simulink model "KinarmStroopTask_260119"  (R2019b)
settings: Solver=ode4  StartTime=0.0  StopTime=inf  FixedStep=BKIN_STEP_TIME  RelTol=1e-3  EnableMultiTasking=on
StartFcn:
  |  warndlg('Dexterit-E models cannot run under simulation. Please compile your model and run it from within Dexterit-E.');set_param(bdroot,'SimulationCommand','stop')
model workspace (MAT data in the model file):
  BKIN_KINEMATIC_FRAME_SIZE = 400
  BKIN_STEP_TIME = 0.00025
  COLOUR_1 = 6
  COLOUR_2 = 7
  COLOUR_3 = 8
  COLOUR_4 = 9
  COLOUR_5 = 10
  E_CONG = 16
  E_CORRECT = 22
  E_FALSE_START = 28
  E_FIX_OFF = 33
  E_FIX_ON = 32
  E_INCONG = 17
  E_INCORRECT = 24
  E_NO_EVENT = 0
  E_REACHED_BLUE = 25
  E_REACHED_GREEN = 26
  E_REACHED_RED = 23
  E_REACHED_T1 = 18
  E_REACHED_T2 = 19
  E_REACHED_T3 = 20
  E_REACHED_T4 = 21
  E_REACHED_YELLOW = 27
  E_SCOL_BLUE = 13
  E_SCOL_GREEN = 14
  E_SCOL_RED = 12
  E_SCOL_YELLOW = 15
  E_STEXT_BLUE = 9
  E_STEXT_GREEN = 10
  E_STEXT_RED = 8
  E_STEXT_YELLOW = 11
  E_STROOP_OFF = 31
  E_T1_ON = 4
  E_T2_ON = 5
  E_T3_ON = 6
  E_T4_ON = 7
  E_TIMED_OUT = 29
  E_TRIAL_END = 30
  E_TRIAL_START = 3
  FIX_DELAY = 12
  FIX_ON_TIME = 11
  FIX_RAND = 13
  FIX_TARG_COL = 4
  FLICKER_ON = 9
  FLICKER_TIME = 10
  LENGTH = 3
  LOAD_X = 1
  LOAD_Y = 2
  PERTURB_SET = 9
  POSTRESP_DELAY = 3
  RADIUS_VIS = 3
  RAMP_DURATION = 4
  RAND_TEXTLOC = 8
  REACH_DELAY = 1
  REACH_RAND = 6
  REACH_TO = 7
  RESULT_TARG_COL = 3
  START_TARG_COL = 2
  STROKE_WIDTH = 13
  STROOP_TARG_COL = 1
  STROOP_USE = 5
  TARG_LENGTH = 3
  TARG_WIDTH = 4
  TEXT = 11
  TEXT1_TARG_COL = 5
  TEXT2_TARG_COL = 6
  TEXT3_TARG_COL = 7
  TEXT4_TARG_COL = 8
  TEXTCIRCLE_MOVE = 14
  TEXTSHOW_DELAY = 2
  TEXT_SIZE = 12
  WIDTH = 4
  Width = 4
  X_LENGTH = 4
  Y_LENGTH = 5
  col_x = 1
  col_y = 2
undefined symbols (not defined in the file or in its folder): slselsubs
libraries: Video x9, General x3, KINARM_general x2, KINARM_EP_loads x2
settings Model: ModifiedComment=chris -- Wed Feb 16 09:18:30 2005 -- Version 1.1384  ModifiedHistory=Feb 16/05 - Add error repeat, add offset ramp  ExtModeArmWhenConnect=off  ExtModeLogAll=off  OrderedModelArguments=off  Creator=Chris Grebeldinger  LastModifiedBy=apark2
settings SolverCC: AutoInsertRateTranBlk=on
settings DataIOCC: SaveFormat=Array  SignalLoggingSaveFormat=ModelDataLogs  SaveOutput=off  SaveTime=off  ReturnWorkspaceOutputs=off  SignalLoggingName=sigsOut
settings OptimizationCC: BlockReduction=off  BooleanDataType=off  OptimizeBlockIOStorage=off  BufferReuse=off  GlobalBufferReuse=off  ExpressionFolding=off  ExpressionDepthLimit=2147483647  LocalBlockOutputs=off  InitFltsAndDblsToZero=on  LifeSpan=inf  OptimizeDataStoreBuffers=off  BusAssignmentInplaceUpdate=off
settings DebuggingCC: SaveWithParameterizedLinksMsg=none  UnderspecifiedInitializationDetection=Classic  MergeDetectMultiDrivingBlocksExec=none  SignalResolutionControl=TryResolveAllWithWarning  MultiTaskDSMMsg=warning  FcnCallInpInsideContextMsg=warning  BusObjectLabelMismatch=none  StateNameClashWarn=warning  StrictBusMsg=ErrorOnBusTreatedAsVector  SFUnexpectedBacktrackingDiag=warning  SFNoUnconditionalDefaultTransitionDiag=warning  SFExecutionAtInitializationDiag=none  ArithmeticOperatorsInVariantConditions=warning
settings HardwareCC: ProdBitPerPointer=32  ProdBitPerSizeT=32  ProdBitPerPtrDiffT=32  ProdLargestAtomicFloat=None  ProdWordSize=32  ProdLongLongMode=on  ProdHWDeviceType=Generic->32-bit x86 compatible  TargetLongLongMode=on  TargetIntDivRoundTo=Zero  TargetEndianess=LittleEndian  TargetHWDeviceType=Generic->32-bit x86 compatible
settings ModelReferenceCC: PropagateSignalLabelsOutOfModel=off
settings SFSimCC: SimCustomHeaderCode="#include \"stdlib.h\""  SimUseLocalCustomCode=off  SimParseCustomCode=off  CustomCodeUndefinedFunction=UseInterfaceOnly
settings RTWCC: Description=Simulink Real-Time  SystemTargetFile=slrt.tlc  TemplateMakefile=slrt_default_tmf  RTWUseLocalCustomCode=off  CustomSourceCode="#include \"stdlib.h\""  CodeExecutionProfiling=on
settings CodeAppCC: MaxIdLength=63  StateflowObjectComments=on
settings SimulinkRealTimeCC: TargetFcnLib=ansi_tfl_tmw.mat  GeneratePreprocessorConditionals=Disable all  PreserveStateflowLocalDataDimensions=off
settings ConfigComp: CovMetricSettings=dw  CovHtmlReporting=on  CovSaveCumulativeToWorkspaceVar=on  CovSaveSingleToWorkspaceVar=on  CovExternalEMLEnable=off

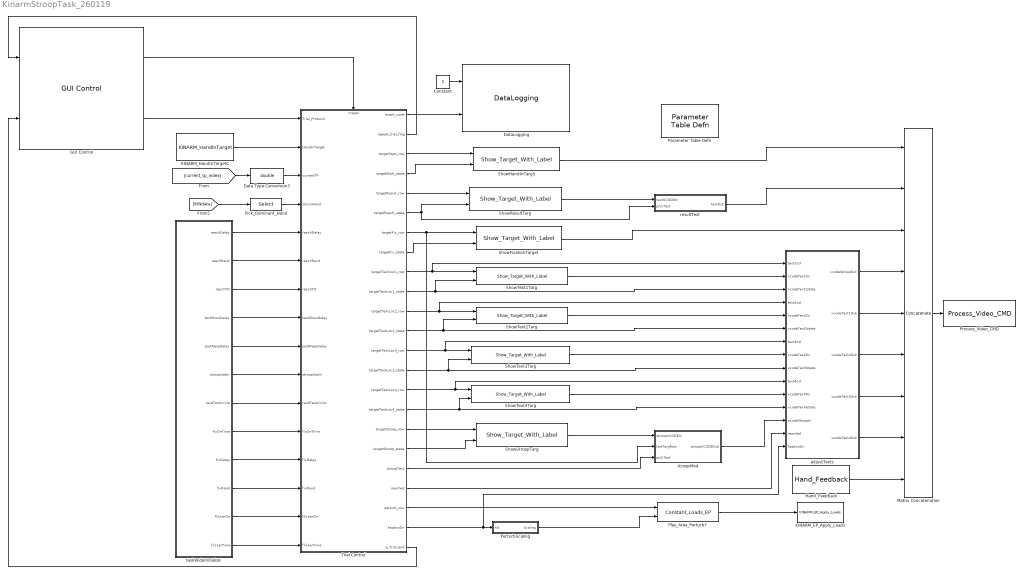
== system KinarmStroopTask_260119 ==
  Constant : Constant
  Data Type Conversion3 : DataTypeConversion  OutDataTypeStr=double
  DataLogging : General/DataLogging  log_event_codes=on  log_analog_inputs=off  show_time_remaining=off  ecat_include=on
  GUI Control : General/GUI Control  task_version=1.0  show_repeat_trial_flag=on  use_custom_tp=off  target_type_str=Circle  Target_Type=1  XYcols=[1 2]  Vcols=3  Lcols=4  indices_padding=[0 0 0 0;0 0 0 0]  target_table_rows=64  load_table_rows=20  tp_table_rows=100
  Hand_Feedback : KINARM_general/Hand_Feedback  feedback_cntl_src=none
  KINARM_EP_Apply_Loads : KINARM_EP_loads/KINARM_EP_Apply_Loads  up_duration=1500  down_duration=1500  max_force=30
  KINARM_HandInTargetC : KINARM_general/KINARM_HandInTarget  use_dominant_hand=on  target_type=Circle  num_states=1  attribcol1=[RADIUS_VIS]  attribcol2=[0]  attribcol3=[0]  attribcol4=[0]  attribcol5=[0]
  Matrix Concatenation : Concatenate  NumInputs=9  Mode=Multidimensional array
  Parameter Table Defn : General/Parameter Table Defn  ShowInLibBrowser=0
  PerturbScaling : Subsystem  mask(Perturbation){}
  Pick_Dominant_Hand : Selector  NumberOfDimensions=2  InputPortWidth=3  IndexOptions=Index vector (dialog),Index vector (dialog)  Indices=[3],[1]  OutputSizes=slselsubs([(-2),(-2)],1),slselsubs([(-2),(-2)],2)
  Play_Area_PerturbY : KINARM_EP_loads/Constant_Loads_EP  use_dom_hand=on  loadcol=[LOAD_X LOAD_Y]  source=port  scaling=1  use_LH_coord=on
  Process_Video_CMD : Video/Process_Video_CMD  video_delay=50
  ShowFixationTarget : Video/Show_Target_With_Label  target_type=Circle  num_states=1  attribcol1=[0 0 0 RADIUS_VIS TEXT COLOUR_1 TEXT_SIZE]  attribcol2=[0 0 0 0 0 0 0]  attribcol3=[0 0 0 0 0 0 0]  attribcol4=[0 0 0 0 0 0 0]  attribcol5=[0 0 0 0 0 0 0]  stateindices_padding=[0 0 0 0;0 0 0 0;0 0 0 0;0 0 0 0;0 0 0 0]  source=dialog  opacity=100  target_display=Both subject and operator displays
  ShowHandInTargS : Video/Show_Target_With_Label  target_type=Circle  num_states=1  attribcol1=[0 COLOUR_1 STROKE_WIDTH RADIUS_VIS 0 0 0]  attribcol2=[0 0 0 0 0 0 0]  attribcol3=[0 0 0 0 0 0 0]  attribcol4=[0 0 0 0 0 0 0]  attribcol5=[0 0 0 0 0 0 0]  stateindices_padding=[0 0 0 0;0 0 0 0;0 0 0 0;0 0 0 0;0 0 0 0]  source=dialog  opacity=100  target_display=Both subject and operator displays
  ShowResultTarg : Video/Show_Target_With_Label  target_type=Circle  num_states=4  attribcol1=[0 0 0 0 TEXT COLOUR_2 TEXT_SIZE]  attribcol2=[0 0 0 0 TEXT COLOUR_1 TEXT_SIZE]  attribcol3=[0 0 0 0 TEXT COLOUR_1 TEXT_SIZE]  attribcol4=[0 0 0 0 TEXT COLOUR_1 TEXT_SIZE]  attribcol5=[0 0 0 0 0 0 0]  stateindices_padding=[0 0 0 0;0 0 0 0;0 0 0 0;0 0 0 0;0 0 0 0]  source=dialog  opacity=100  target_display=Both subject and operator displays
  ShowStroopTarg : Video/Show_Target_With_Label  target_type=Rectangle  num_states=4  attribcol1=[COLOUR_5 0 0 0 0 0 0 COLOUR_1 TEXT_SIZE]  attribcol2=[COLOUR_5 0 0 0 0 0 0 COLOUR_2 TEXT_SIZE]  attribcol3=[COLOUR_5 0 0 0 0 0 0 COLOUR_3 TEXT_SIZE]  attribcol4=[COLOUR_5 0 0 0 0 0 0 COLOUR_4 TEXT_SIZE]  attribcol5=[0 0 0 0 0 0 0 0 0]  stateindices_padding=[0 0;0 0;0 0;0 0;0 0]  source=dialog  opacity=100  target_display=Both subject and operator displays
  ShowText1Targ : Video/Show_Target_With_Label  target_type=Circle  num_states=4  attribcol1=[0 COLOUR_1 STROKE_WIDTH RADIUS_VIS TEXT COLOUR_1 TEXT_SIZE]  attribcol2=[0 COLOUR_1 STROKE_WIDTH RADIUS_VIS TEXT COLOUR_1 TEXT_SIZE]  attribcol3=[0 COLOUR_1 STROKE_WIDTH RADIUS_VIS TEXT COLOUR_1 TEXT_SIZE]  attribcol4=[0 COLOUR_1 STROKE_WIDTH RADIUS_VIS TEXT COLOUR_1 TEXT_SIZE]  attribcol5=[0 0 0 0 0 0 0]  stateindices_padding=[0 0 0 0;0 0 0 0;0 0 0 0;0 0 0 0;0 0 0 0]  source=dialog  opacity=100  target_display=Both subject and operator displays
  ShowText2Targ : Video/Show_Target_With_Label  target_type=Circle  num_states=4  attribcol1=[0 COLOUR_1 STROKE_WIDTH RADIUS_VIS TEXT COLOUR_1 TEXT_SIZE]  attribcol2=[0 COLOUR_1 STROKE_WIDTH RADIUS_VIS TEXT COLOUR_1 TEXT_SIZE]  attribcol3=[0 COLOUR_1 STROKE_WIDTH RADIUS_VIS TEXT COLOUR_1 TEXT_SIZE]  attribcol4=[0 COLOUR_1 STROKE_WIDTH RADIUS_VIS TEXT COLOUR_1 TEXT_SIZE]  attribcol5=[0 0 0 0 0 0 0]  stateindices_padding=[0 0 0 0;0 0 0 0;0 0 0 0;0 0 0 0;0 0 0 0]  source=dialog  opacity=100  target_display=Both subject and operator displays
  ShowText3Targ : Video/Show_Target_With_Label  target_type=Circle  num_states=4  attribcol1=[0 COLOUR_1 STROKE_WIDTH RADIUS_VIS TEXT COLOUR_1 TEXT_SIZE]  attribcol2=[0 COLOUR_1 STROKE_WIDTH RADIUS_VIS TEXT COLOUR_1 TEXT_SIZE]  attribcol3=[0 COLOUR_1 STROKE_WIDTH RADIUS_VIS TEXT COLOUR_1 TEXT_SIZE]  attribcol4=[0 COLOUR_1 STROKE_WIDTH RADIUS_VIS TEXT COLOUR_1 TEXT_SIZE]  attribcol5=[0 0 0 0 0 0 0]  stateindices_padding=[0 0 0 0;0 0 0 0;0 0 0 0;0 0 0 0;0 0 0 0]  source=dialog  opacity=100  target_display=Both subject and operator displays
  ShowText4Targ : Video/Show_Target_With_Label  target_type=Circle  num_states=4  attribcol1=[0 COLOUR_1 STROKE_WIDTH RADIUS_VIS TEXT COLOUR_1 TEXT_SIZE]  attribcol2=[0 COLOUR_1 STROKE_WIDTH RADIUS_VIS TEXT COLOUR_1 TEXT_SIZE]  attribcol3=[0 COLOUR_1 STROKE_WIDTH RADIUS_VIS TEXT COLOUR_1 TEXT_SIZE]  attribcol4=[0 COLOUR_1 STROKE_WIDTH RADIUS_VIS TEXT COLOUR_1 TEXT_SIZE]  attribcol5=[0 0 0 0 0 0 0]  stateindices_padding=[0 0 0 0;0 0 0 0;0 0 0 0;0 0 0 0;0 0 0 0]  source=dialog  opacity=100  target_display=Both subject and operator displays
  Trial Control : Stateflow chart  TreatAsAtomicUnit=on
  adjustTexts : Subsystem
  resultText : Subsystem
  stroopMod : Subsystem
  taskWideInitialize : Subsystem
  wires:
  Trial Control/23(e_Trial_End) -> GUI Control/2
  Matrix Concatenation/1 -> Process_Video_CMD/1
  Trial Control/1(event_code) -> DataLogging/2
  Constant/1 -> DataLogging/1
  GUI Control/2 -> Trial Control/1(Trial_Protocol)
  Trial Control/2(repeat_trial_flag) -> GUI Control/1
  [current_tp_index] -> Data Type Conversion3/1
  ShowResultTarg/1 -> resultText/1(textVCODEIn)
  KINARM_HandInTargetC/1 -> Trial Control/2(HandInTarget)
  Hand_Feedback/1 -> Matrix Concatenation/9
  GUI Control/1 -> Trial Control/Trigger
  Data Type Conversion3/1 -> Trial Control/3(currentTP)
  stroopMod/1(stroopVCODEOut) -> adjustTexts/13(vcodeStroopIn)
  Trial Control/16(targetTextLoc4_state) -> adjustTexts/12(vcodeText4state), ShowText4Targ/2
  Trial Control/15(targetTextLoc4_row) -> ShowText4Targ/1, adjustTexts/10("text4col ")
  Trial Control/14(targetTextLoc3_state) -> ShowText3Targ/2, adjustTexts/9(vcodeText3state)
  Trial Control/13(targetTextLoc3_row) -> adjustTexts/7(text3col), ShowText3Targ/1
  Trial Control/11(targetTextLoc2_row) -> ShowText2Targ/1, adjustTexts/4(text2col)
  Trial Control/9(targetTextLoc1_row) -> adjustTexts/1(text1col), ShowText1Targ/1
  Trial Control/10(targetTextLoc1_state) -> adjustTexts/3(vcodeText1state), ShowText1Targ/2
  Trial Control/5(targetResult_row) -> ShowResultTarg/1
  Trial Control/6(targetResult_state) -> resultText/2(pickText), ShowResultTarg/2
  Trial Control/17(targetStroop_row) -> ShowStroopTarg/1
  Trial Control/18(targetStroop_state) -> ShowStroopTarg/2
  taskWideInitialize/1(reachDelay) -> Trial Control/5(reachDelay)
  taskWideInitialize/2(reachRand) -> Trial Control/6(reachRand)
  taskWideInitialize/5(postRespDelay) -> Trial Control/9(postRespDelay)
  ShowStroopTarg/1 -> stroopMod/1(stroopVCODEIn)
  Trial Control/12(targetTextLoc2_state) -> adjustTexts/6(vcodeText2state), ShowText2Targ/2
  ShowText1Targ/1 -> adjustTexts/2(vcodeText1In)
  ShowText2Targ/1 -> adjustTexts/5(vcodeText2In)
  ShowText3Targ/1 -> adjustTexts/8(vcodeText3In)
  ShowText4Targ/1 -> adjustTexts/11(vcodeText4In)
  resultText/1(textOut) -> Matrix Concatenation/2
  Trial Control/19(stroopText) -> stroopMod/3(pickText)
  Trial Control/20(reached) -> adjustTexts/14(reached)
  adjustTexts/2(vcodeText1Out) -> Matrix Concatenation/5
  adjustTexts/3(vcodeText2Out) -> Matrix Concatenation/6
  adjustTexts/4(vcodeText3Out) -> Matrix Concatenation/7
  adjustTexts/5(vcodeText4Out) -> Matrix Concatenation/8
  Play_Area_PerturbY/1 -> KINARM_EP_Apply_Loads/1
  PerturbScaling/1(Scaling) -> Play_Area_PerturbY/2
  Trial Control/22(hapticsOn) -> adjustTexts/15(hapticsOn), PerturbScaling/1(hit)
  Trial Control/21(perturb_row) -> Play_Area_PerturbY/1
  adjustTexts/1("vcodeStroopOut ") -> Matrix Concatenation/4
  Trial Control/3(targetStart_row) -> ShowHandInTargS/1
  Trial Control/4(targetStart_state) -> ShowHandInTargS/2
  ShowHandInTargS/1 -> Matrix Concatenation/1
  taskWideInitialize/6(stroopUseIn) -> Trial Control/10(stroopUseIn)
  taskWideInitialize/3(reachTO) -> Trial Control/7(reachTO)
  taskWideInitialize/4(textShowDelay) -> Trial Control/8(textShowDelay)
  taskWideInitialize/7(randTextcircle) -> Trial Control/11(randTextcircle)
  taskWideInitialize/11(flickerOn) -> Trial Control/15(flickerOn)
  taskWideInitialize/12(flickerTime) -> Trial Control/16(flickerTime)
  taskWideInitialize/8(fixOnTime) -> Trial Control/12(fixOnTime)
  taskWideInitialize/9(fixDelay) -> Trial Control/13(fixDelay)
  taskWideInitialize/10(fixRand) -> Trial Control/14(fixRand)
  Trial Control/7(targetFix_row) -> stroopMod/2(lastTargRow), ShowFixationTarget/1
  Trial Control/8(targetFix_state) -> ShowFixationTarget/2
  ShowFixationTarget/1 -> Matrix Concatenation/3
  [KINdata] -> Pick_Dominant_Hand/1
  Pick_Dominant_Hand/1 -> Trial Control/4(whichHand)

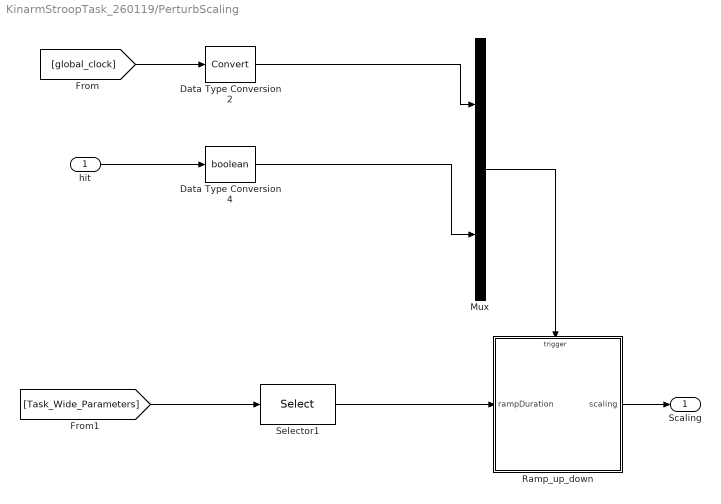
== system KinarmStroopTask_260119/PerturbScaling ==
  hit : Inport
  Data Type Conversion2 : DataTypeConversion
  Data Type Conversion4 : DataTypeConversion  OutDataTypeStr=boolean
  Mux : Mux  Inputs=2
  Ramp_up_down : Stateflow chart  TreatAsAtomicUnit=on
  Selector1 : Selector  NumberOfDimensions=2  InputPortWidth=3  IndexOptions=Index vector (dialog),Select all  Indices=[RAMP_DURATION],[3]  OutputSizes=slselsubs([(-2),(-2)],1),1
  Scaling : Outport  VectorParamsAs1DForOutWhenUnconnected=off
  wires:
  Ramp_up_down/1(scaling) -> Scaling/1
  [global_clock] -> Data Type Conversion2/1
  Data Type Conversion2/1 -> Mux/1
  [Task_Wide_Parameters] -> Selector1/1
  Selector1/1 -> Ramp_up_down/1(rampDuration)
  Mux/1 -> Ramp_up_down/Trigger
  hit/1 -> Data Type Conversion4/1
  Data Type Conversion4/1 -> Mux/2

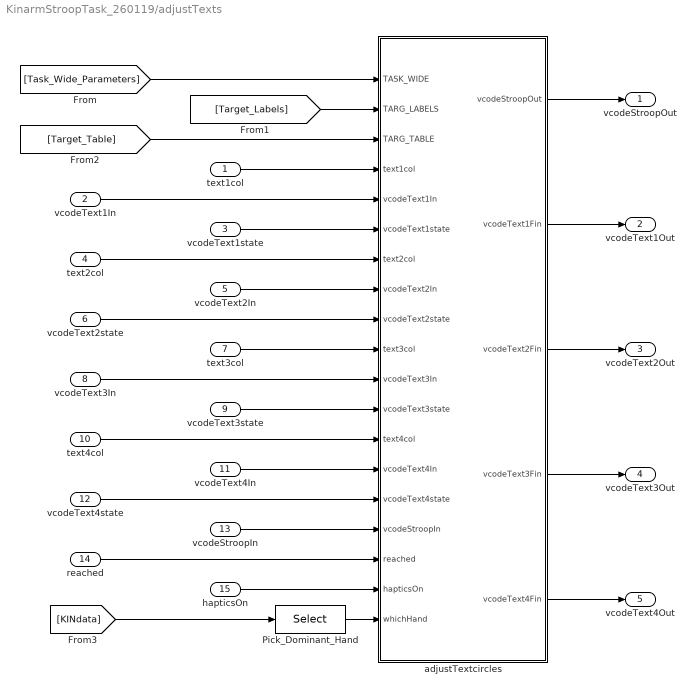
== system KinarmStroopTask_260119/adjustTexts ==
  text1col : Inport
  vcodeText1In : Inport  Port=2
  vcodeText1state : Inport  Port=3
  text2col : Inport  Port=4
  vcodeText2In : Inport  Port=5
  vcodeText2state : Inport  Port=6
  text3col : Inport  Port=7
  vcodeText3In : Inport  Port=8
  vcodeText3state : Inport  Port=9
  "text4col " : Inport  Port=10
  vcodeText4In : Inport  Port=11
  vcodeText4state : Inport  Port=12
  vcodeStroopIn : Inport  Port=13
  reached : Inport  Port=14
  hapticsOn : Inport  Port=15
  Pick_Dominant_Hand : Selector  NumberOfDimensions=2  InputPortWidth=3  IndexOptions=Index vector (dialog),Index vector (dialog)  Indices=[3],[1]  OutputSizes=slselsubs([(-2),(-2)],1),slselsubs([(-2),(-2)],2)
  "adjustTextcircles " : MATLAB Function  TreatAsAtomicUnit=on
  "vcodeStroopOut " : Outport
  vcodeText1Out : Outport  Port=2
  vcodeText2Out : Outport  Port=3
  vcodeText3Out : Outport  Port=4
  vcodeText4Out : Outport  Port=5
  wires:
  hapticsOn/1 -> "adjustTextcircles "/18(hapticsOn)
  "adjustTextcircles "/2(vcodeText1Fin) -> vcodeText1Out/1
  vcodeText1In/1 -> "adjustTextcircles "/5(vcodeText1In)
  vcodeText2In/1 -> "adjustTextcircles "/8(vcodeText2In)
  "adjustTextcircles "/3(vcodeText2Fin) -> vcodeText2Out/1
  "adjustTextcircles "/4(vcodeText3Fin) -> vcodeText3Out/1
  vcodeText4In/1 -> "adjustTextcircles "/14(vcodeText4In)
  vcodeText3In/1 -> "adjustTextcircles "/11(vcodeText3In)
  reached/1 -> "adjustTextcircles "/17(reached)
  "adjustTextcircles "/5(vcodeText4Fin) -> vcodeText4Out/1
  [Task_Wide_Parameters] -> "adjustTextcircles "/1(TASK_WIDE)
  vcodeStroopIn/1 -> "adjustTextcircles "/16(vcodeStroopIn)
  vcodeText1state/1 -> "adjustTextcircles "/6(vcodeText1state)
  vcodeText2state/1 -> "adjustTextcircles "/9(vcodeText2state)
  vcodeText3state/1 -> "adjustTextcircles "/12(vcodeText3state)
  vcodeText4state/1 -> "adjustTextcircles "/15(vcodeText4state)
  "adjustTextcircles "/1(vcodeStroopOut) -> "vcodeStroopOut "/1
  [Target_Labels] -> "adjustTextcircles "/2(TARG_LABELS)
  [Target_Table] -> "adjustTextcircles "/3(TARG_TABLE)
  text1col/1 -> "adjustTextcircles "/4(text1col)
  text2col/1 -> "adjustTextcircles "/7(text2col)
  text3col/1 -> "adjustTextcircles "/10(text3col)
  "text4col "/1 -> "adjustTextcircles "/13(text4col)
  [KINdata] -> Pick_Dominant_Hand/1
  Pick_Dominant_Hand/1 -> "adjustTextcircles "/19(whichHand)

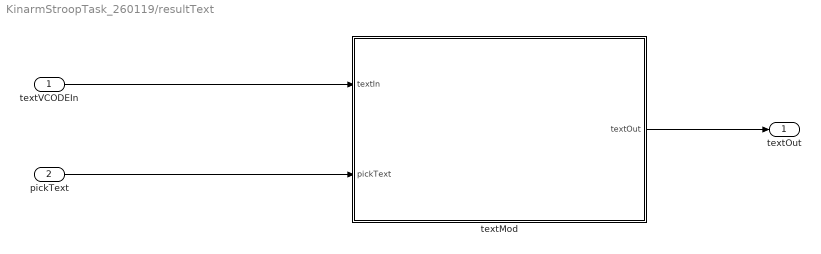
== system KinarmStroopTask_260119/resultText ==
  textVCODEIn : Inport
  pickText : Inport  Port=2
  textMod : MATLAB Function  TreatAsAtomicUnit=on
  textOut : Outport
  wires:
  textMod/1(textOut) -> textOut/1
  textVCODEIn/1 -> textMod/1(textIn)
  pickText/1 -> textMod/2(pickText)

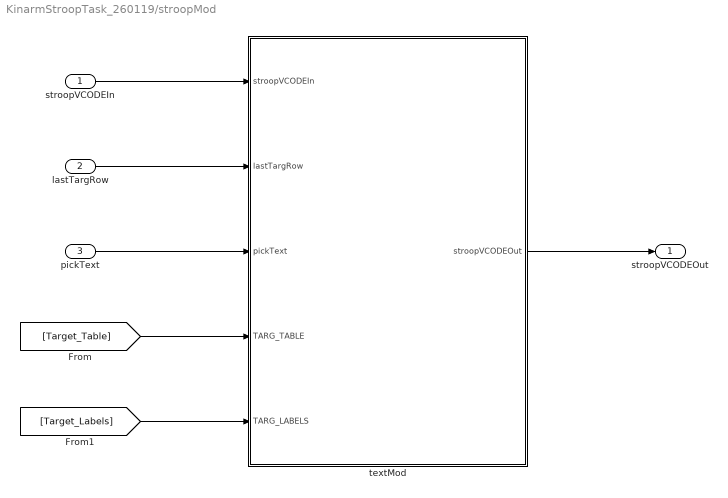
== system KinarmStroopTask_260119/stroopMod ==
  stroopVCODEIn : Inport
  lastTargRow : Inport  Port=2
  pickText : Inport  Port=3
  textMod : MATLAB Function  TreatAsAtomicUnit=on
  stroopVCODEOut : Outport
  wires:
  textMod/1(stroopVCODEOut) -> stroopVCODEOut/1
  stroopVCODEIn/1 -> textMod/1(stroopVCODEIn)
  pickText/1 -> textMod/3(pickText)
  [Target_Table] -> textMod/4(TARG_TABLE)
  [Target_Labels] -> textMod/5(TARG_LABELS)
  lastTargRow/1 -> textMod/2(lastTargRow)

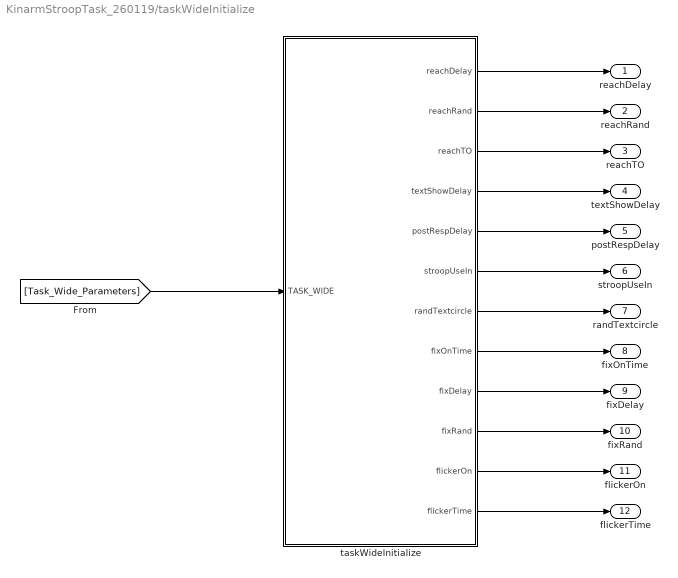
== system KinarmStroopTask_260119/taskWideInitialize ==
  taskWideInitialize : MATLAB Function  TreatAsAtomicUnit=on
  reachDelay : Outport
  reachRand : Outport  Port=2
  reachTO : Outport  Port=3
  textShowDelay : Outport  Port=4
  postRespDelay : Outport  Port=5
  stroopUseIn : Outport  Port=6
  randTextcircle : Outport  Port=7
  fixOnTime : Outport  Port=8
  fixDelay : Outport  Port=9
  fixRand : Outport  Port=10
  flickerOn : Outport  Port=11
  flickerTime : Outport  Port=12
  wires:
  [Task_Wide_Parameters] -> taskWideInitialize/1(TASK_WIDE)
  taskWideInitialize/1(reachDelay) -> reachDelay/1
  taskWideInitialize/2(reachRand) -> reachRand/1
  taskWideInitialize/4(textShowDelay) -> textShowDelay/1
  taskWideInitialize/5(postRespDelay) -> postRespDelay/1
  taskWideInitialize/6(stroopUseIn) -> stroopUseIn/1
  taskWideInitialize/3(reachTO) -> reachTO/1
  taskWideInitialize/7(randTextcircle) -> randTextcircle/1
  taskWideInitialize/12(flickerTime) -> flickerTime/1
  taskWideInitialize/11(flickerOn) -> flickerOn/1
  taskWideInitialize/8(fixOnTime) -> fixOnTime/1
  taskWideInitialize/9(fixDelay) -> fixDelay/1
  taskWideInitialize/10(fixRand) -> fixRand/1

== matlab function KinarmStroopTask_260119/adjustTexts/adjustTextcircles  ==
  data: vcodeStroopOut output; TASK_WIDE input; TARG_LABELS input; TARG_TABLE input; text1col input; vcodeText1In input; vcodeText1state input; text2col input; vcodeText2In input; vcodeText2state input; text3col input; vcodeText3In input; vcodeText3state input; text4col input; vcodeText4In input; vcodeText4state input; vcodeStroopIn input; reached input; vcodeText1Fin output; vcodeText2Fin output; vcodeText3Fin output; vcodeText4Fin output; hapticsOn input; whichHand input; POSTRESP_DELAY parameter; BKIN_STEP_TIME parameter; TEXT parameter; TEXTCIRCLE_MOVE parameter
function [vcodeStroopOut, vcodeText1Fin, vcodeText2Fin, vcodeText3Fin, vcodeText4Fin] = fcn...
    (TASK_WIDE, TARG_LABELS, TARG_TABLE, text1col, vcodeText1In, vcodeText1state, text2col, vcodeText2In, vcodeText2state,...
    text3col, vcodeText3In, vcodeText3state, text4col, vcodeText4In, vcodeText4state, vcodeStroopIn, reached, hapticsOn,whichHand,...
    POSTRESP_DELAY, BKIN_STEP_TIME, TEXT, TEXTCIRCLE_MOVE)
%this function modifies the textcircle's movement (if reached correctly) and
%text using the target table
%stroop vcode is routed through this function just for cleaner simulink

%initialize taskwides
postReachDelay = TASK_WIDE(POSTRESP_DELAY); %time after reach completed
textcircleMove = TASK_WIDE(TEXTCIRCLE_MOVE); %turn on or off the Textcircles moving
dt = BKIN_STEP_TIME;
speedScalar = 1000/postReachDelay;

%set output vcodes
vcodeStroopOut = vcodeStroopIn;
vcodeText1Out = vcodeText1In;
vcodeText2Out = vcodeText2In;
vcodeText3Out = vcodeText3In;
vcodeText4Out = vcodeText4In;

%set up textcircle movement
persistent atTime0 moveDistX moveDistY
if (isempty(atTime0))
    atTime0 = 0;
    moveDistX = 0;
    moveDistY = 0;
end

if (hapticsOn == 1 && textcircleMove == 1) %if reach is correct move the textcircle towards the stroop target
    if (reached == 1) %if textcircle1 is reached
        moveDistX = moveDistX + dt*(vcodeStroopIn(1,3)-vcodeText1Out(1,3))*speedScalar; %move the textcircle in the xdirection
        moveDistY = moveDistY + dt*(vcodeStroopIn(1,4)-vcodeText1Out(1,4))*speedScalar; %move the textcircle in the ydirection
        vcodeText1Out(1,3) = vcodeText1Out(1,3)+moveDistX;
        vcodeText1Out(1,4) = vcodeText1Out(1,4)+moveDistY;
    elseif (reached == 2) %if textcircle2 is reached
        moveDistX = moveDistX + dt*(vcodeStroopIn(1,3)-vcodeText2Out(1,3))*speedScalar;
        moveDistY = moveDistY + dt*(vcodeStroopIn(1,4)-vcodeText2Out(1,4))*speedScalar;
        vcodeText2Out(1,3) = vcodeText2Out(1,3)+moveDistX;
        vcodeText2Out(1,4) = vcodeText2Out(1,4)+moveDistY;
    elseif (reached == 3) %if textcircle3 is reached
        moveDistX = moveDistX + dt*(vcodeStroopIn(1,3)-vcodeText3Out(1,3))*speedScalar;
        moveDistY = moveDistY + dt*(vcodeStroopIn(1,4)-vcodeText3Out(1,4))*speedScalar;
        vcodeText3Out(1,3) = vcodeText3Out(1,3)+moveDistX;
        vcodeText3Out(1,4) = vcodeText3Out(1,4)+moveDistY;
    elseif (reached == 4) %if textcircle4 is reached
        moveDistX = moveDistX + dt*(vcodeStroopIn(1,3)-vcodeText4Out(1,3))*speedScalar;
        moveDistY = moveDistY + dt*(vcodeStroopIn(1,4)-vcodeText4Out(1,4))*speedScalar;
        vcodeText4Out(1,3) = vcodeText4Out(1,3)+moveDistX;
        vcodeText4Out(1,4) = vcodeText4Out(1,4)+moveDistY;
    end
end

if (reached == 0) %reset the movement
    atTime0 = [];
end

%% text mod

%modify the textcircle texts based on the target table and input from
%stateflow
%text can be changed to accomodate for language change but should not be
%changed to a different colour (i.e position 1 must be red, rouge, etc...)
%changing it to a different colour will not let the task operate properly
%as position 1 (far-left position) will always represent red
vcodeText1Fin = textMod(vcodeText1Out,vcodeText1state,TARG_LABELS,TARG_TABLE,TEXT,text1col,text2col,text3col,text4col,whichHand);
vcodeText2Fin = textMod(vcodeText2Out,vcodeText2state,TARG_LABELS,TARG_TABLE,TEXT,text1col,text2col,text3col,text4col,whichHand);
vcodeText3Fin = textMod(vcodeText3Out,vcodeText3state,TARG_LABELS,TARG_TABLE,TEXT,text1col,text2col,text3col,text4col,whichHand);
vcodeText4Fin = textMod(vcodeText4Out,vcodeText4state,TARG_LABELS,TARG_TABLE,TEXT,text1col,text2col,text3col,text4col,whichHand);

function textVCODEOut = textMod(textVCODEIn,textVCODEstate,TARG_LABELS,TARG_TABLE,TEXT,text1col,text2col,text3col,text4col,whichHand)
%modify the label target to display appropriate text
textCircle1 = TARG_LABELS(TARG_TABLE(text1col,TEXT),1:10); %modify text1 based on input row from stateflow
textCircle2 = TARG_LABELS(TARG_TABLE(text2col,TEXT),1:10);
textCircle3 = TARG_LABELS(TARG_TABLE(text3col,TEXT),1:10);
textCircle4 = TARG_LABELS(TARG_TABLE(text4col,TEXT),1:10);

    textVCODEOut = textVCODEIn;
    if (textVCODEstate == 1) %red text
        str1 = uint16(textCircle1);
    elseif (textVCODEstate == 2) %blue text
        str1 = uint16(textCircle2);
    elseif (textVCODEstate == 3) %green text
        str1 = uint16(textCircle3);
    elseif (textVCODEstate == 4) %yellow text
        str1 = uint16(textCircle4);
    else
        str1 = uint16(['Error']);
    end
    if (whichHand == 2) %if the hand is left then flip the texts (far left <=> far right, mid left <=> mid right)
        if (textVCODEstate == 1) %red text
            str1 = uint16(textCircle4);
        elseif (textVCODEstate == 2) %blue text
            str1 = uint16(textCircle3);
        elseif (textVCODEstate == 3) %green text
            str1 = uint16(textCircle2);
        elseif (textVCODEstate == 4) %yellow text
            str1 = uint16(textCircle1);
        else
            str1 = uint16(['Error']);
        end
    end
    textVCODEOut(1,15:(length(str1)+14))=(str1);  %str in letters
end
end

== stateflow chart KinarmStroopTask_260119/Trial Control ==
  state flipForHand/
    %swap left and right targets to accomodate for left hand
    targetTextLoc1_row = Trial_Protocol(TEXT4_TARG_COL); %show far left Textcircle
    targetTextLoc2_row = Trial_Protocol(TEXT3_TARG_COL); %show mid left Textcircle
    targetTextLoc3_row = Trial_Protocol(TEXT2_TARG_COL); %show mid right Textcircle
    targetTextLoc4_row = Trial_Protocol(TEXT1_TARG_COL); %show far right Textcircle
  state Initialize/
    %setup the variables
    targetStart_row = Trial_Protocol(START_TARG_COL); %get Start Target
    targetResult_row = Trial_Protocol(RESULT_TARG_COL); %Result Target shows error text
    targetFix_row = Trial_Protocol(FIX_TARG_COL); %fixation target
    targetStroop_row = Trial_Protocol(STROOP_TARG_COL); %get Stroop Target
    targetTextLoc1_row = Trial_Protocol(TEXT1_TARG_COL); %show far left Textcircle
    targetTextLoc2_row = Trial_Protocol(TEXT2_TARG_COL); %show mid left Textcircle
    targetTextLoc3_row = Trial_Protocol(TEXT3_TARG_COL); %show mid right Textcircle
    targetTextLoc4_row = Trial_Protocol(TEXT4_TARG_COL); %show far right Textcircle
    perturb_row = Trial_Protocol(PERTURB_SET); %get the perturbation row
    targetStart_state = 0; %turn off Start Target
    targetResult_state = 0; %turn off Result Text
    targetFix_state = 0; %turn off fixation target
    targetStroop_state = 0; %turn off Stroop Target
    targetTextLoc1_state = 0; %turn off one Textcircle
    targetTextLoc2_state = 0; %turn off one Textcircle
    targetTextLoc3_state = 0; %turn off one Textcircle
    targetTextLoc4_state = 0; %turn off one Textcircle
    hapticsOn = 0; %no haptic feedback
    reached = 0; %outputs the Textcircle reached
    whichCol = 0; %which colour is is reached (1=red,2=blue,3=green,4=yellow)
    trialCount = 0; %count the trials
    randArray = randperm(24); %set up a random array that is persistent through task
    stroopUse = 0; %which variant is used (1=50,50,2=25,75,3=congOnly, 4=incongOnly, 4
    %is also used for neutral blocks but the text needs to change to neutral as well)
  state MainTrial
    state startTrial/
      %get the Stroop text/colour and Textcircle order and show Start Target
      entry:
      targetStart_state = 1;
      trialCount = trialCount + 1;
      [stroopState,stroopText, textOut] = pickPairs(currentTP,randArray(currentTP),stroopUse,randTextcircle);
      randReach = reachRand*rand();
      randFix = fixRand*rand();
      event_code = E_TRIAL_START;
    state stroopTextEvents/
      state stroopTRed/
        event_code = E_STEXT_RED;
      state stroopTBlue/
        event_code = E_STEXT_BLUE;
      state stroopTGreen/
        event_code = E_STEXT_GREEN;
      state stroopTYellow/
        event_code = E_STEXT_YELLOW;
    state stroopAppear/
      %show Stroop Target
      targetStart_state = 0;
      targetStroop_state = stroopState;
    state falseStart/
      %left Start Target too early
      event_code = E_FALSE_START;
      targetResult_state = 4;
      targetTextLoc1_state = 0;
      targetTextLoc2_state = 0;
      targetTextLoc3_state = 0;
      targetTextLoc4_state = 0;
      targetFix_state = 0;
    state reset/
      targetResult_state = 0;
    state nice1/
      %looks nice
    state displayTextcircles
      %sequentially show the textcircles and exit state if hand leaves the start target (delay should be minimum 1 to show event code)
      state FixOn/
        %show fixation Target
        targetFix_state = 1;
        event_code = E_FIX_ON;
      state startText1/
        %show first Textcircle
        targetTextLoc1_state = textOut(1,1);
        event_code = E_T1_ON;
      state startText4/
        %show fourth Textcircle
        targetTextLoc4_state = textOut(4,1);
        event_code = E_T4_ON;
      state FixOff/
        %turn off fixation Target
        targetFix_state = 0;
        event_code = E_FIX_OFF;
      state startText3/
        %show third Textcircle
        targetTextLoc3_state =  textOut(3,1);
        event_code = E_T3_ON
      state startText2/
        %show second Textcircle
        targetTextLoc2_state = textOut(2,1);
        event_code = E_T2_ON;
      FixOn -> FixOff : after(fixOnTime,msec)
      startText4 -> FixOn : %wait for delay to show Stroop Target
          | after(randReach+reachDelay,msec)
      startText1 -> startText2 : %after a time
          | after(textShowDelay,msec)
      startText3 -> startText4 : %after a time
          | after(textShowDelay,msec)
      startText2 -> startText3 : %after a time
          | after(textShowDelay,msec)
    state stroopColourEvents/
      state stroopCRed/
        event_code = E_SCOL_RED;
      state stroopCBlue/
        event_code = E_SCOL_BLUE;
      state stroopCGreen/
        event_code = E_SCOL_GREEN;
      state stroopCYellow/
        event_code = E_SCOL_YELLOW;
    state nice2/
    state nice4/
    state textcircleReachedEvents/
      state reached1/
        %Textcircle1 reached and save state
        event_code = E_REACHED_T1;
        whichCol = targetTextLoc1_state;
        reached = 1;
      state reached2/
        %Textcircle2 reached and save state
        event_code = E_REACHED_T2;
        whichCol = targetTextLoc2_state;
        reached = 2;
      state reached3/
        %Textcircle3 reached and save state
        event_code = E_REACHED_T3;
        whichCol = targetTextLoc3_state;
        reached = 3;
      state reached4/
        %Textcircle4 reached and save state
        event_code = E_REACHED_T4;
        whichCol = targetTextLoc4_state;
        reached = 4;
    state nice3/
    state trialType/
      state cong/
        %event code for
        %congruent trials
        event_code = E_CONG;
      state incong/
        %event code for
        %incongruent trials
        event_code = E_INCONG;
    state flickering/
      targetStroop_state = 0;
      event_code = E_STROOP_OFF;
    state timeoutTrial/
      %didnt reach a Textcircle
      event_code = E_TIMED_OUT;
      targetResult_state = 3;
      targetStart_state = 0;
    state reachedColourEvents/
      state redReach/
        %send out colour of the textcircle reached
        event_code = E_REACHED_RED;
      state blueReach/
        %send out colour of the textcircle reached
        event_code = E_REACHED_BLUE;
      state greenReach/
        %send out colour of the textcircle reached
        event_code = E_REACHED_GREEN;
      state yellowReach/
        %send out colour of the textcircle reached
        event_code = E_REACHED_YELLOW;
    state nice5/
    state trialResultEvents/
      state correct/
        %reach to Textcircle was correct
        %and turn on haptic feedback
        hapticsOn = 1;
        event_code = E_CORRECT;
      state incorrect/
        %reach to Textcircle was incorrect
        %and show text on screen
        event_code = E_INCORRECT;
        targetResult_state = 2;
    state trialEnd/
      %turn off all targets
      event_code = E_TRIAL_END;
      targetResult_state = 0;
      targetStroop_state = 0;
      targetTextLoc1_state = 0;
      targetTextLoc2_state = 0;
      targetTextLoc3_state = 0;
      targetTextLoc4_state = 0;
      hapticsOn = 0;
    stroopAppear -> stroopTRed [order 1] : %Stroop text is red
        | [stroopText == 1]
    stroopAppear -> stroopTBlue [order 4] : %Stroop text is blue
        | [stroopText == 2]
    stroopAppear -> stroopTGreen [order 3] : %Stroop text is green
        | [stroopText == 3]
    startTrial -> reset
    stroopAppear -> stroopTYellow [order 2] : %Stroop text is yellow
        | [stroopText == 4]
    (junction 701) -> reset : after(postRespDelay/2,msec)
    falseStart -> (junction 701) : %check hand in Start Target
        | [HandInTarget(targetStart_row) == 1]
    displayTextcircles -> falseStart : %hand left the Start Target
        | [HandInTarget(targetStart_row) == 0]
    reset -> startText1 : %check hand in Start Target
        | [HandInTarget(targetStart_row) == 1]
    stroopTextEvents -> nice1 : after(1,msec)
    FixOff -> stroopAppear : after(fixDelay+randFix,msec)
    nice1 -> stroopCYellow [order 4] : %Stroop colour is yellow
        | [stroopState == 4]
    nice1 -> stroopCGreen [order 3] : %Stroop colour is green
        | [stroopState == 3]
    nice1 -> stroopCBlue [order 2] : %Stroop colour is blue
        | [stroopState == 2]
    nice1 -> stroopCRed [order 1] : %Stroop colour is red
        | [stroopState == 1]
    stroopColourEvents -> nice2 : after(1,msec)
    nice2 -> cong [order 1] : %Stroop colour and text are congruent
        | [stroopState == stroopText]
    nice2 -> incong [order 2] : %Stroop colour and text
        | %are incongruent
    reached1 -> nice4 [order 1] : %reached Textcircle1 correctly
        | [targetTextLoc1_state == stroopState]
    nice3 -> reached1 [order 1] : %hand into Textcircle1
        | [HandInTarget(targetTextLoc1_row)==1]
    trialType -> nice3 [order 2] : [flickerOn ==0]
    reached1 -> incorrect [order 2] : after(1,msec)
    reached2 -> nice4 [order 1] : %reached Textcircle2 correctly
        | [targetTextLoc2_state == stroopState]
    trialType -> (junction 696) [order 1] : [flickerOn == 1]
    nice3 -> reached2 [order 2] : %hand into Textcircle2
        | [HandInTarget(targetTextLoc2_row)==1]
    reached2 -> incorrect [order 2] : after(1,msec)
    reached3 -> nice4 [order 1] : %reached Textcircle3 correctly
        | [targetTextLoc3_state == stroopState]
    (junction 696) -> flickering : after(flickerTime,msec)
    nice3 -> reached3 [order 3] : %hand into Textcircle3
        | [HandInTarget(targetTextLoc3_row)==1]
    flickering -> nice3 : after(1,msec)
    reached3 -> incorrect [order 2] : after(1,msec)
    reached4 -> nice4 [order 1] : %reached Textcircle4 correctly
        | [targetTextLoc4_state == stroopState]
    nice3 -> reached4 [order 4] : %hand into Textcircle4
        | [HandInTarget(targetTextLoc4_row)==1]
    nice3 -> timeoutTrial [order 5] : %didnt reach in time
        | after(reachTO,msec)
    nice4 -> correct : after(1,msec)
    reached4 -> incorrect [order 2] : after(1,msec)
    timeoutTrial -> trialEnd : %show result text until next trial
        | after(postRespDelay,msec)
    nice5 -> redReach [order 1] : %reached Textcircle was red
        | [whichCol == 1]
    nice5 -> blueReach [order 2] : %reached Textcircle was blue
        | [whichCol == 2]
    trialResultEvents -> nice5 : after(1,msec)
    nice5 -> greenReach [order 3] : %reached Textcircle was green
        | [whichCol == 3]
    reachedColourEvents -> trialEnd : %intertrial delay
        | after(postRespDelay,msec)
    nice5 -> yellowReach [order 4] : %reached Textcircle was yellow
        | [whichCol == 4]
  state showInstruction/
    %show Instruction Image
    targetStart_state = 1;
    stroopUse = stroopUseIn;
    targetResult_state = 1;
  state Inter_Trial_State/
    %turn off all
    entry:
    event_code = 0;
    repeat_trial_flag = 0;
    reached = 0;
    hapticsOn = 0;
    whichCol = 0;
    targetStart_state = 0;
    targetResult_state = 0;
    targetStroop_state = 0;
    targetTextLoc1_state = 0;
    targetTextLoc2_state = 0;
    targetTextLoc3_state = 0;
    targetTextLoc4_state = 0;
    e_Trial_End;
  state RepeatTrial/
    entry:
    repeat_trial_flag = 1;
  state resetTrialCount/
    %get new random perm after 24 trials
    entry:
    randArray = randperm(24);
    trialCount = 0;
  (default) -> Initialize
  (junction 719) -> flipForHand [order 1] : %left hand
      | [whichHand == 2]
  flipForHand -> showInstruction
  showInstruction -> startTrial : %check hand in Start Target
      | [HandInTarget(targetStart_row) == 1]
  Initialize -> (junction 719) : %wait for task to start
      | [currentTP > 0]
  (junction 719) -> showInstruction [order 2] : %right hand
      | [whichHand == 1]
  Inter_Trial_State -> startTrial [order 1] : after(1,msec)
  RepeatTrial -> Inter_Trial_State : after(1,msec)
  MainTrial -> RepeatTrial : e_ExitTrialNow
      | % e_ExitTrialNow event occurs if the
      | % Dex pause is pressed by the operator
  resetTrialCount -> Inter_Trial_State
  Inter_Trial_State -> resetTrialCount [order 2] : %check if all trial types used
      | [trialCount == 24]
  trialEnd -> Inter_Trial_State : after(1,msec)
  data: stateStroop function_output; textNumStroop function_output; outText function_output; nowTP function_input; randTP function_input; useStroop function_input; textcircleRand function_input; event_code output [0..]; repeat_trial_flag output; targetStart_row output; targetStart_state output; Trial_Protocol input; HandInTarget input; targetResult_row output; targetResult_state output; targetFix_row output; targetFix_state output; targetTextLoc1_row output; targetTextLoc1_state output; targetTextLoc2_row output; targetTextLoc2_state output; targetTextLoc3_row output; targetTextLoc3_state output; targetTextLoc4_row output; targetTextLoc4_state output; targetStroop_row output; targetStroop_state output; stroopText output; reached output; perturb_row output; hapticsOn output; currentTP input; whichHand input; reachDelay input; reachRand input; reachTO input; textShowDelay input; postRespDelay input; stroopState local; textOut local; whichCol local; trialCount local; randArray local; stroopUseIn input; stroopUse local; randReach local; randTextcircle input; fixOnTime input; fixDelay input; fixRand input; flickerOn input; flickerTime input; randFix local
  events: e_clk input RISING_EDGE_EVENT; e_ExitTrialNow input RISING_EDGE_EVENT; e_Trial_End output EITHER_EDGE_EVENT
  function [stateStroop,textNumStroop,outText] = pickPairs(nowTP,randTP,useStroop,textcircleRand):
    | function [stateStroop,textNumStroop,outText] = pickPairs(nowTP,randTP,useStroop,textcircleRand)
    | %This function sets up an array for the Stroop Target pairs (text-colour) 
    | %using a combination of 4 texts (red,blue,green,yellow) and 4 
    | %colours = 16 combinations (i.e. red text, blue colour). Normally these 
    | %pairs would have 25% congruent/75% incongruent trials. To reduce the heavy 
    | %bias of incongruent trials, 8 additional congruent trials (red-red, 
    | %blue-blue, etc...) were added to achieve 50% congruent/incongruent trials
    | %for a total of 24 trials.
    | %This function also setups up an array to get the location of the 4 
    | %Textcircles to reach for (location-text pairs: location 1 text box = 
    | %red, location 2 = blue, 3 = green, 4 = yellow). There are a total of 24 
    | %combinations based on 4 different texts in 4 different locations. 
    | %To achieve an equal number of all Stroop Target pairs and all Textcircle 
    | %pairs, each block of trials must be 24 trials in length.
    | %1 = red
    | %2 = blue
    | %3 = green
    | %4 = yellow
    | 
    | %useStroop is set in the taskwide params
    | %% set up random arrays for Stroop Target colour-text pairs and location-text pairs
    | 
    | %50% congruent/incongruent array for Stroop Target colour-text pairs
    | stroopArrayEven = [1 2 3 4 1 2 3 4 1 2 3 4 1 2 3 4 1 2 3 4 1 2 3 4;... %row is colours
    |                    1 1 1 1 2 2 2 2 3 3 3 3 4 4 4 4 1 2 3 4 1 2 3 4;];  %row is texts
    | %25%/75% congruent/incongruent
    | stroopArrayQuart = [1 2 3 4 1 2 3 4 1 2 3 4 1 2 3 4 1 2 3 4 1 2 3 4;... %row is colours
    |                     1 1 1 1 2 2 2 2 3 3 3 3 4 4 4 4 1 1 2 2 3 3 4 4;];  %row is texts
    | %all congruent (blocked stroop)
    | stroopArrayCong = [1 2 3 4 1 2 3 4 1 2 3 4 1 2 3 4 1 2 3 4 1 2 3 4;...
    |                    1 2 3 4 1 2 3 4 1 2 3 4 1 2 3 4 1 2 3 4 1 2 3 4];
    | %all incongruent (blocked stroop)
    | stroopArrayIncong = [1 2 3 4 1 2 3 4 1 2 3 4 1 2 3 4 1 2 3 4 1 2 3 4;...
    |                      2 3 4 1 3 4 2 1 3 4 1 2 4 1 2 3 2 3 4 1 3 4 1 2;];
    | 
    | %24 groups of 4 location-text pairs for the textcircles (any colour can be
    | %in any location)
    | locTextArrayRand = [1 1 1 1 1 1 2 2 2 2 2 2 3 3 3 3 3 3 4 4 4 4 4 4; %text of textcircle 1 in position1 (row represents position (1-far left, 2-mid left, 3-mid right, 4-far right), number represents colour)
    |                     2 2 3 3 4 4 1 1 3 3 4 4 1 1 2 2 4 4 1 1 2 2 3 3; %text of textcircle 2 in position2 
    |                     3 4 2 4 2 3 3 4 1 4 1 3 2 4 1 4 1 2 2 3 1 3 1 2; %text of textcircle 3 in position3 
    |                     4 3 4 2 3 2 4 3 4 1 3 1 4 2 4 1 2 1 3 2 3 1 2 1];%text of textcircle 4 in position4 
    | 
    | %colours are fixed to their position (1-far left = red, 2-mid left = blue, 3-mid right = green, 4-far right = yellow)                
    | locTextArray = [1 1 1 1 1 1 1 1 1 1 1 1 1 1 1 1 1 1 1 1 1 1 1 1; %text of textcircle 1 in position1 
    |                 2 2 2 2 2 2 2 2 2 2 2 2 2 2 2 2 2 2 2 2 2 2 2 2; %text of textcircle 2 in position2
    |                 3 3 3 3 3 3 3 3 3 3 3 3 3 3 3 3 3 3 3 3 3 3 3 3; %text of textcircle 3 in position3
    |                 4 4 4 4 4 4 4 4 4 4 4 4 4 4 4 4 4 4 4 4 4 4 4 4];%text of textcircle 4 in position4
    |             
    | %% output variables
    | if (useStroop == 2) %use 25,75 variant
    |     stroopArrayUse = stroopArrayQuart;
    | elseif (useStroop == 3) %use only congruent (blocked stroop)
    |     stroopArrayUse = stroopArrayCong;
    | elseif (useStroop == 4) %use only incongruent/neutral (blocked stroop)
    |     stroopArrayUse = stroopArrayIncong;
    | else %use 50,50 variant
    |     stroopArrayUse = stroopArrayEven;
    | end
    | 
    | %get a random column of the arrow based on randTP
    | stateStroop = stroopArrayUse(1,randTP); %stroop colour pulled by random value from randTP
    | textNumStroop = stroopArrayUse(2,randTP); %stroop text pulled by random value from randTP
    | 
    | %grabs the values for Textcircles
    | if (textcircleRand == 1) %random colour in each position
    |     outText = locTextArrayRand(:,nowTP); %Textcircle only randomized by Dex so TP#1-24 will be associated with a specific sequence later in data analysis
    | else %fixed colour in each position
    |     outText = locTextArray(:,nowTP); %Textcircle location is not randomized
    | end

== matlab function KinarmStroopTask_260119/taskWideInitialize/taskWideInitialize ==
  data: TASK_WIDE input; reachDelay output; reachRand output; reachTO output; textShowDelay output; postRespDelay output; REACH_DELAY parameter; REACH_RAND parameter; TEXTSHOW_DELAY parameter; REACH_TO parameter; POSTRESP_DELAY parameter; stroopUseIn output; STROOP_USE parameter; randTextcircle output; fixOnTime output; fixDelay output; fixRand output; RAND_TEXTLOC parameter; flickerOn output; flickerTime output; FLICKER_ON parameter; FLICKER_TIME parameter; FIX_DELAY parameter; FIX_ON_TIME parameter; FIX_RAND parameter
function [reachDelay, reachRand, reachTO, textShowDelay, postRespDelay, stroopUseIn, randTextcircle, fixOnTime, fixDelay, fixRand, flickerOn, flickerTime] =...
    fcn(TASK_WIDE, REACH_DELAY, REACH_RAND, TEXTSHOW_DELAY, REACH_TO, POSTRESP_DELAY, STROOP_USE, RAND_TEXTLOC, FLICKER_ON, FLICKER_TIME, FIX_DELAY, FIX_ON_TIME, FIX_RAND)  

%% task wide parameter outputs
reachDelay = TASK_WIDE(REACH_DELAY); %time for holding hand in Start Target
reachRand = TASK_WIDE(REACH_RAND); %random time added to reachDelay
reachTO = TASK_WIDE(REACH_TO); %time to reach for a textbox
textShowDelay = TASK_WIDE(TEXTSHOW_DELAY); %time between textbox appearances
postRespDelay = TASK_WIDE(POSTRESP_DELAY); %time between trials
stroopUseIn = TASK_WIDE(STROOP_USE); %gets the variant of stroop to use 50/50 or 25/75 congruent/incongruent
randTextcircle = TASK_WIDE(RAND_TEXTLOC); %turn on (1) or off (0) textcircle location randomization
fixOnTime = TASK_WIDE(FIX_ON_TIME); %time the fixation cross stays on
fixDelay = TASK_WIDE(FIX_DELAY); %time after fixation cross turns off
fixRand = TASK_WIDE(FIX_RAND); %random time added to fixation delay
flickerOn = TASK_WIDE(FLICKER_ON); %feature to turn on (1) or off (0) the ability to turn off the Stroop early
flickerTime = TASK_WIDE(FLICKER_TIME); %time the Stroop stays on for

== matlab function KinarmStroopTask_260119/stroopMod/textMod ==
  data: stroopVCODEIn input; lastTargRow input; pickText input; stroopVCODEOut output; TARG_TABLE input; TEXT parameter; TARG_LABELS input
function stroopVCODEOut  = fcn(stroopVCODEIn, lastTargRow, pickText, TARG_TABLE, TEXT, TARG_LABELS)
%function modifies the stroop target to read in text from unused targets

%starts at Target position #fixation+1 which should be unused
stroopText1 = TARG_LABELS(TARG_TABLE(lastTargRow+1,TEXT),1:10); 
stroopText2 = TARG_LABELS(TARG_TABLE(lastTargRow+2,TEXT),1:10);
stroopText3 = TARG_LABELS(TARG_TABLE(lastTargRow+3,TEXT),1:10);
stroopText4 = TARG_LABELS(TARG_TABLE(lastTargRow+4,TEXT),1:10);

%set the output text based on stroopText
stroopVCODEOut = stroopVCODEIn;
if (pickText == 1) %text in TT row after fixation cross
    str1 = uint16(stroopText1);
elseif (pickText == 2) %text in TT row after fixation cross
    str1 = uint16(stroopText2);
elseif (pickText == 3) %text in TT row after fixation cross
    str1 = uint16(stroopText3);
elseif (pickText == 4) %text in TT row after fixation cross
    str1 = uint16(stroopText4);
else
    str1 = uint16(['Error']);
end
stroopVCODEOut(1,15:(length(str1)+14))= (str1);  %str in letters

== matlab function KinarmStroopTask_260119/resultText/textMod ==
  data: textIn input; pickText input; textOut output
function textOut  = fcn(textIn, pickText)
%function modifies the trial result text with hardcoded text

textOut = textIn;
if (pickText == 1) %text for beginning the task
    str1 = ['Place your cursor inside the circle to begin'];
elseif (pickText == 2) %incorrect trials output
    str1 = ['Incorrect!'];
elseif (pickText == 3) %timed out trials output
    str1 = ['Too slow!'];
elseif (pickText == 4) %false start trials output
    str1 = ['Stay in the circle!'];
else %checks errors
    str1 = ['Error'];
end
textOut(1,15:(length(str1)+14))=uint16(str1);  %str in letters

== stateflow chart KinarmStroopTask_260119/PerturbScaling/Ramp_up_down ==
  state peak/
    entry: scaling=1;
  state RampingUp/
    entry: tick=0;
    CurrScale=scaling;
    b=rampDuration/2; % Center at Middle;
    c=rampDuration/10; % Define Rise Rate;
    during:
    tick++;
    scaling = (1-CurrScale)/(1+exp(-1*(tick-b)/c))+CurrScale;
  state RampingDown/
    entry: tick=0;
    CurrScale=scaling;
    b=rampDuration/2; % Center at Middle;
    c=rampDuration/10; % Define Drop Rate;
    during:
    tick++;
    scaling = CurrScale*(1-1/(1+exp(-1*(tick-b)/c)));
  state minimum/
    entry: scaling=0;
  RampingUp -> peak : after(rampDuration, e_clk)
  peak -> RampingDown
  RampingDown -> minimum : after(rampDuration, e_clk)
  minimum -> RampingUp : e_hit/
  (default) -> minimum
  data: rampDuration input double; scaling output double; tick local double; c local double; b local double; CurrScale local double
  events: e_clk input RISING_EDGE_EVENT; e_hit input RISING_EDGE_EVENT
